simulink model "LQR_simulation"  (R2023b)
settings: Solver=VariableStepAuto  StartTime=0.0  StopTime=30  RelTol=1e-3
values from neighbouring files (symbols this model uses):
  A = [0 1 0 0;32.79 0 6.625 0;0 0 0 1;-67.38 0 -8.92 0]    [LQR.m]
  AobsK = kalmf.A    [LQR.m]
  B = [0 0; 4.65 -7.94;0 0;-7.94 27.27]    [LQR.m]
  BobsK = kalmf.B    [LQR.m]
  C = [1 0 0 0;0 0 1 0]    [LQR.m]
  D = zeros(2,2)    [LQR.m]
  gainMatrix = dcgain(transferFunctionPos^-1)    [LQR.m]
  gainMatrixa = dcgain(transferFunctionPosa^-1)    [LQR.m]
  Qtilde = diag(Qtildeelements)    [LQR.m]
  Rtilde = diag(Rtildeelements)    [LQR.m]
undefined symbols (not defined in the file or in its folder): Continuous, K, Ka, Ki, Time
libraries: simulink x6, ctrlSharedLib x1
settings Model: Creator=Giammo  LastModifiedBy=Giammo

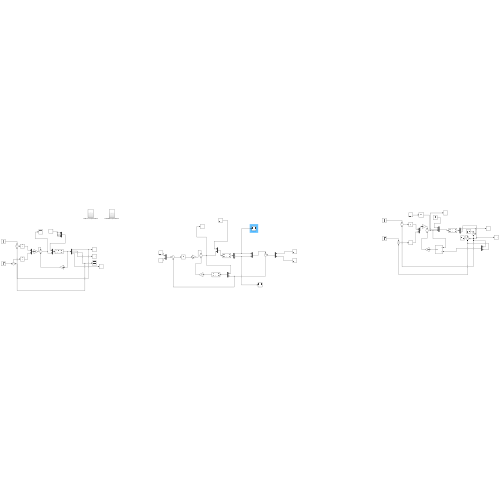
[thumbnail: Simulink's stored preview of the top-level diagram]
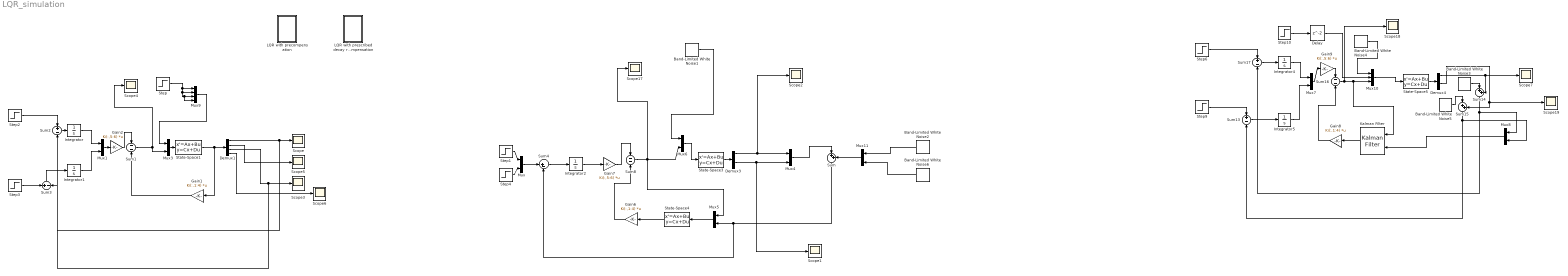
== system LQR_simulation ==
  Band-Limited White Noise1 : simulink/Sources/Band-Limited White Noise  Cov=diag(Qtilde)*1e-3  Ts=1e-3  seed=[23341]
  Band-Limited White Noise2 : simulink/Sources/Band-Limited White Noise  Cov=Rtilde(1,1)*1e-3  Ts=1e-3  seed=[23341]
  Band-Limited White Noise3 : simulink/Sources/Band-Limited White Noise  Cov=Rtilde(1,1)*1e-3  Ts=1e-3  seed=[23341]
  Band-Limited White Noise4 : simulink/Sources/Band-Limited White Noise  Cov=diag(Qtilde)*1e-3  Ts=1e-3  seed=[23341]
  Band-Limited White Noise5 : simulink/Sources/Band-Limited White Noise  Cov=Rtilde(2,2)*1e-3  Ts=1e-3  seed=[23341]
  Band-Limited White Noise6 : simulink/Sources/Band-Limited White Noise  Cov=Rtilde(1,1)*1e-3  Ts=1e-3  seed=[23341]
  Delay : Delay
  Demux1 : Demux
  Demux3 : Demux
  Demux4 : Demux
  Gain1 : Gain  Gain=Ki(:,1:4)  Multiplication=Matrix(K*u)
  Gain2 : Gain  Gain=Ki(:,5:6)  Multiplication=Matrix(K*u)
  Gain6 : Gain  Gain=Ki(:,1:4)  Multiplication=Matrix(K*u)
  Gain7 : Gain  Gain=Ki(:,5:6)  Multiplication=Matrix(K*u)
  Gain8 : Gain  Gain=Ki(:,1:4)  Multiplication=Matrix(K*u)
  Gain9 : Gain  Gain=Ki(:,5:6)  Multiplication=Matrix(K*u)
  Integrator{,1..2,4..5} (5 alike) : Integrator
  Kalman Filter : ctrlSharedLib/Kalman Filter  TimeDomain=Continuous-Time  UseCurrentEstimator=on  ModelSource=Individual A, B, C, D matrices  ModelSourceVariable=ss(0.95,1,1,0,1)  A=A  B=B  C=C  D=D  NumberOfStates=1  NumberOfInputs=1  NumberOfOutputs=1  InitialEstimateSource=Dialog  X0=[0.5;0;0;0]  P0=10  UseK=off  UseGH=off  NumberOfProcessNoiseInputs=1  G=1  TimeInvariantG=on  H=0  TimeInvariantH=on  Q=diag(Qtilde)*1e-3  TimeInvariantQ=on  R=diag(Rtilde)*1e-3  TimeInvariantR=on  N=0  TimeInvariantN=on  AddInputPort=on  AddEnablePort=off  OutputEstimatedY=off  OutputP=off  Ts=-1
  LQR with precompensation : Subsystem
  LQR with prescribed decay rate and precompensation : Subsystem
  Mux{,1,3..8,11} (9 alike) : Mux  Inputs=2
  Mux10 : Mux  Inputs=3
  Mux9 : Mux
  Scope{,1..7,17..19} (11 alike) : Scope
  State-Space1 : StateSpace  A=A  B=[eye(4) B]  C=eye(4)  D=zeros(4,6)  InitialCondition=0
  State-Space3 : StateSpace  A=A  B="[eye(4)  B]"  C=eye(4)  D=zeros(4,6)  InitialCondition=0
  State-Space4 : StateSpace  A=AobsK  B=BobsK  C=eye(4,4)  D=zeros(4,4)  InitialCondition=[0.2;0;0.1;0]
  State-Space5 : StateSpace  A=A  B=[[1 0 0 0 1;0 1 0 0 1;0 0 1 0 1;0 0 0 1 1] B]  C=eye(4)  D=zeros(4,7)  InitialCondition=0
  Step : Step  After=0.5  SampleTime=0
  Step{1..4,6,9} (6 alike) : Step  After=0.26  SampleTime=0
  Step10 : Step  After=0  SampleTime=0
  Sum : Sum  Inputs=|++
  Sum1 : Sum  Inputs=--
  Sum{2..3,13,17} (4 alike) : Sum  Inputs=+-
  Sum14 : Sum  Inputs=|++
  Sum15 : Sum  Inputs=|++
  Sum16 : Sum  Inputs=--
  Sum4 : Sum  Inputs=|+-
  Sum8 : Sum  Inputs=--
  wires:
  Gain1/1 -> Sum1/2
  Demux1/3 -> Sum3/2, Scope3/1
  Demux1/1 -> Scope/1, Sum2/2
  State-Space1/1 -> Gain1/1, Demux1/1
  Sum2/1 -> Integrator/1
  Step2/1 -> Sum2/1
  Step3/1 -> Sum3/1
  Sum3/1 -> Integrator1/1
  Integrator/1 -> Mux1/1
  Integrator1/1 -> Mux1/2
  Mux1/1 -> Gain2/1
  Gain2/1 -> Sum1/1
  Demux1/2 -> Scope5/1
  Demux1/4 -> Scope6/1
  Sum1/1 -> Mux3/2, Scope4/1
  Gain7/1 -> Sum8/1
  State-Space3/1 -> Demux3/1
  State-Space4/1 -> Gain6/1
  Gain6/1 -> Sum8/2
  Mux5/1 -> State-Space4/1
  Mux6/1 -> State-Space3/1
  Band-Limited White Noise1/1 -> Mux6/1
  Demux4/3 -> Scope19/1, Sum15/2
  Sum15/1 -> Mux8/2, Sum13/2
  Sum14/1 -> Mux8/1, Sum17/2
  Band-Limited White Noise5/1 -> Sum15/1
  Band-Limited White Noise4/1 -> Mux10/1
  Gain8/1 -> Sum16/2
  Demux4/1 -> Scope7/1, Sum14/2
  Step6/1 -> Sum17/1
  Sum16/1 -> Scope18/1, Mux10/3, Kalman Filter/1
  Sum13/1 -> Integrator5/1
  Mux7/1 -> Gain9/1
  State-Space5/1 -> Demux4/1
  Integrator5/1 -> Mux7/2
  Mux10/1 -> State-Space5/1
  Sum17/1 -> Integrator4/1
  Band-Limited White Noise3/1 -> Sum14/1
  Step9/1 -> Sum13/1
  Integrator4/1 -> Mux7/1
  Gain9/1 -> Sum16/1
  Mux8/1 -> Kalman Filter/2
  Kalman Filter/1 -> Gain8/1
  Step10/1 -> Delay/1
  Delay/1 -> Mux10/2
  Sum8/1 -> Mux5/1, Mux6/2, Scope17/1
  Mux3/1 -> State-Space1/1
  Step/1 -> Mux9/4, Mux9/3, Mux9/2, Mux9/1
  Mux9/1 -> Mux3/1
  Demux3/1 -> Scope2/1, Mux4/1
  Demux3/3 -> Scope1/1, Mux4/2
  Mux4/1 -> Sum/1
  Band-Limited White Noise6/1 -> Mux11/2
  Band-Limited White Noise2/1 -> Mux11/1
  Mux11/1 -> Sum/2
  Sum/1 -> Sum4/2, Mux5/2
  Step1/1 -> Mux/1
  Step4/1 -> Mux/2
  Mux/1 -> Sum4/1
  Sum4/1 -> Integrator2/1
  Integrator2/1 -> Gain7/1

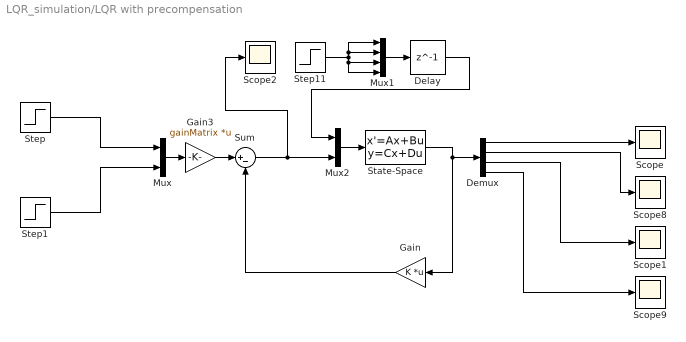
== system LQR_simulation/LQR with precompensation ==
  Delay : Delay  DelayLength=1
  Demux : Demux
  Gain : Gain  Gain=K  Multiplication=Matrix(K*u)
  Gain3 : Gain  Gain=gainMatrix  Multiplication=Matrix(K*u)
  Mux : Mux  Inputs=2
  Mux1 : Mux
  Mux2 : Mux  Inputs=2
  Scope{,1..2,8..9} (5 alike) : Scope
  State-Space : StateSpace  A=A  B=[eye(4) B]  C=eye(4)  D=zeros(4,6)  InitialCondition=0
  Step : Step  After=0.26  SampleTime=0
  Step1 : Step  After=0.26  SampleTime=0
  Step11 : Step  After=0.13  SampleTime=0
  Sum : Sum  Inputs=|+-
  wires:
  Gain/1 -> Sum/2
  Demux/1 -> Scope/1
  Step1/1 -> Mux/2
  Demux/3 -> Scope1/1
  Demux/2 -> Scope8/1
  Step/1 -> Mux/1
  Gain3/1 -> Sum/1
  Mux2/1 -> State-Space/1
  State-Space/1 -> Gain/1, Demux/1
  Demux/4 -> Scope9/1
  Mux/1 -> Gain3/1
  Step11/1 -> Mux1/4, Mux1/3, Mux1/1, Mux1/2
  Sum/1 -> Scope2/1, Mux2/2
  Mux1/1 -> Delay/1
  Delay/1 -> Mux2/1

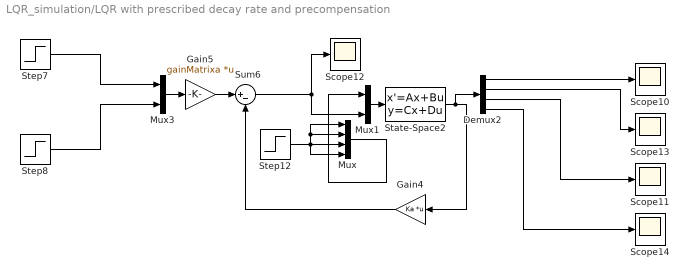
== system LQR_simulation/LQR with prescribed decay rate and precompensation ==
  Demux2 : Demux
  Gain4 : Gain  Gain=Ka  Multiplication=Matrix(K*u)
  Gain5 : Gain  Gain=gainMatrixa  Multiplication=Matrix(K*u)
  Mux : Mux
  Mux1 : Mux  Inputs=2
  Mux3 : Mux  Inputs=2
  Scope{10..14} (5 alike) : Scope
  State-Space2 : StateSpace  A=A  B=[eye(4) B]  C=eye(4)  D=zeros(4,6)  InitialCondition=0
  Step12 : Step  After=0.13  SampleTime=0
  Step7 : Step  After=0.26  SampleTime=0
  Step8 : Step  After=0.26  SampleTime=0
  Sum6 : Sum  Inputs=|+-
  wires:
  Mux3/1 -> Gain5/1
  Demux2/2 -> Scope13/1
  Step7/1 -> Mux3/1
  Gain4/1 -> Sum6/2
  Demux2/1 -> Scope10/1
  Demux2/4 -> Scope14/1
  Gain5/1 -> Sum6/1
  Step8/1 -> Mux3/2
  Demux2/3 -> Scope11/1
  State-Space2/1 -> Gain4/1, Demux2/1
  Sum6/1 -> Mux1/2, Scope12/1
  Step12/1 -> Mux/4, Mux/3, Mux/2, Mux/1
  Mux1/1 -> State-Space2/1
  Mux/1 -> Mux1/1
